simulink model "Controller_test"  (R2025b)
settings: Solver=FixedStepDiscrete  StartTime=0.0  StopTime=3*tHold  FixedStep=Ts  RelTol=1e-3
PreLoadFcn:
  | controller_params
InitFcn:
  | controller_params
undefined symbols (not defined in the file): Ao, Bo, DiscIntNeverNeededParam, K, Ke, plantD, preD, preMap, rLow, tExc, tHold, Ts, uLim, vBias, x0map, xPlant0
libraries: simulink x1
settings Model: Creator=havard  LastModifiedBy=havard

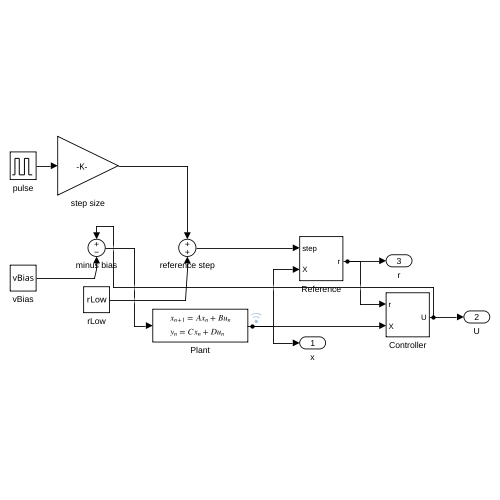
[thumbnail: Simulink's stored preview of the top-level diagram]
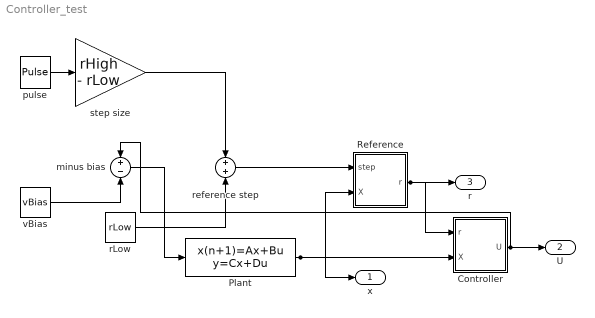
== system Controller_test ==
  Controller : Subsystem
  Plant : DiscreteStateSpace  A=plantD.A  B=plantD.B  C=plantD.C  D=0  InitialCondition=[0; xPlant0; 0; xPlant0; 0]  SampleTime=Ts
  Reference : Subsystem
  minus bias : Sum  Inputs=+-
  pulse : DiscretePulseGenerator  PulseType=Time based  Period=2*tHold  PulseWidth=50  PhaseDelay=tHold
  rLow : Constant  Value=rLow
  reference step : Sum
  step size : Gain  Gain=rHigh - rLow
  vBias : Constant  Value=vBias
  x : Outport
  U : Outport  Port=2
  r : Outport  Port=3
  wires:
  Reference/1(r) -> r/1, Controller/1(r)
  Plant/1 -> x/1, Reference/2(X), Controller/2(X)
  reference step/1 -> Reference/1(step)
  minus bias/1 -> Plant/1
  rLow/1 -> reference step/2
  step size/1 -> reference step/1
  vBias/1 -> minus bias/2
  pulse/1 -> step size/1
  Controller/1(U) -> minus bias/1, U/1

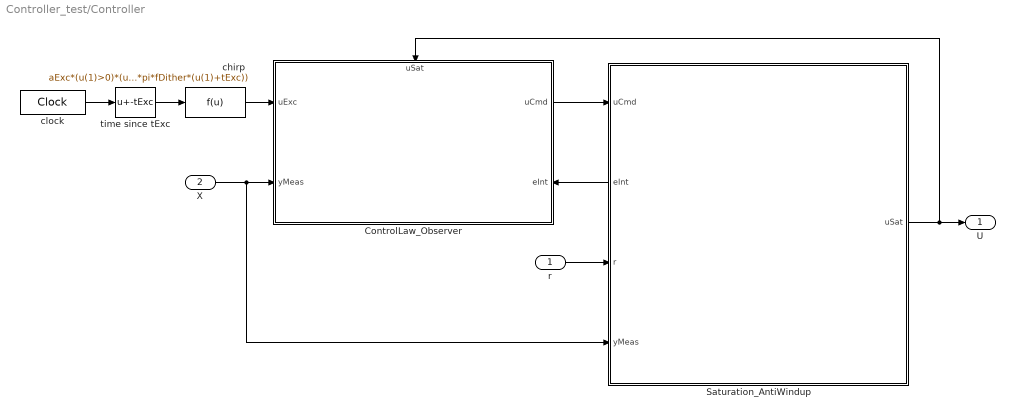
== system Controller_test/Controller ==
  r : Inport
  X : Inport  Port=2
  ControlLaw_Observer : Subsystem
      settings: PortSchema="{\"entries\":[{\"content\":{\"sides\":[{\"content\":{\"connectorIds\":[\"In1\",\"In2\"]},\"type\":\"ConnectorPlacement.EquallySpacedRectSide\",\"uuid\":\"4ab0fcb8-52c7-4a4e-9377-be86be06758b\"},{\"content\":{\"connectorIds\":[\"Out1\",\"In4\"],\"side\":\"RIGHT\"},\"type\":\"ConnectorPlacement.EquallySpacedRectSide\",\"uuid\":\"0c93ed77-db89-4914-8ed3-cc59a8eb3b85\"},{\"content\":{\"connectorIds\":[\"In3\"],\"side\":\"TOP\"},\"type\":\"ConnectorPlacement.EquallySpacedRectSide\",\"uuid\":\"1c748175-366b-4d57-8d03-3856bbcdfb09\"},{\"content\":{\"side\":\"BOTTOM\"},\"type\":\"ConnectorPlacement.EquallySpacedRectSide\",\"uuid\":\"18ee6780-29bb-4133-baad-5bb614cd70f7\"}]},\"type\":\"ConnectorPlacement.EquallySpacedConnector\",\"uuid\":\"9b829baf-7a37-4ed0-ad0c-dec2a53cf1cf\"}],\"packageUris\":[\"http://schema.mathworks.com/mf0/Connector/R2020b\"],\"version\":\"1.0\"}"
  Saturation_AntiWindup : Subsystem
      settings: PortSchema="{\"entries\":[{\"content\":{\"sides\":[{\"content\":{\"connectorIds\":[\"In1\",\"Out2\",\"In2\",\"In3\"]},\"type\":\"ConnectorPlacement.EquallySpacedRectSide\",\"uuid\":\"fd51be67-1b16-4c80-8941-43d479349b34\"},{\"content\":{\"connectorIds\":[\"Out1\"],\"side\":\"RIGHT\"},\"type\":\"ConnectorPlacement.EquallySpacedRectSide\",\"uuid\":\"50a9a10a-2e08-446e-b14e-5678e3c6d1e3\"},{\"content\":{\"side\":\"TOP\"},\"type\":\"ConnectorPlacement.EquallySpacedRectSide\",\"uuid\":\"8fd36ea3-ab38-479f-a719-6e347c4892f4\"}]},\"type\":\"ConnectorPlacement.EquallySpacedConnector\",\"uuid\":\"95e37cf3-826c-49dc-833f-2565447af58e\"}],\"packageUris\":[\"http://schema.mathworks.com/mf0/Connector/R2020b\"],\"version\":\"1.0\"}"
  chirp : Fcn  Expr=aExc*(u(1)>0)*(u(1)<tExcDur)*sin(2*pi*(fExc1*u(1) + (fExc2-fExc1)/(2*tExcDur)*u(1)^2)) + aDither*sin(2*pi*fDither*(u(1)+tExc))
  clock : DigitalClock  SampleTime=Ts
  time since tExc : Bias  Bias=-tExc  SaturateOnIntegerOverflow=off
  U : Outport
  wires:
  time since tExc/1 -> chirp/1
  clock/1 -> time since tExc/1
  chirp/1 -> ControlLaw_Observer/1(uExc)
  Saturation_AntiWindup/2(eInt) -> ControlLaw_Observer/4(eInt)
  Saturation_AntiWindup/1(uSat) -> ControlLaw_Observer/3(uSat), U/1
  ControlLaw_Observer/1(uCmd) -> Saturation_AntiWindup/1(uCmd)
  X/1 -> Saturation_AntiWindup/3(yMeas), ControlLaw_Observer/2(yMeas)
  r/1 -> Saturation_AntiWindup/2(r)

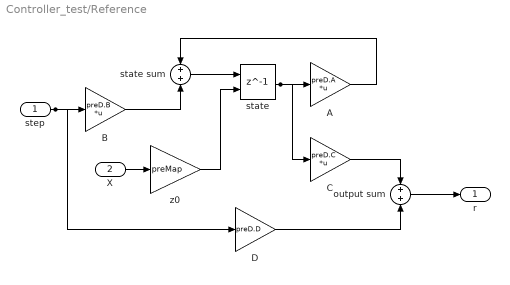
== system Controller_test/Reference ==
  step : Inport
  X : Inport  Port=2
  A : Gain  Gain=preD.A  Multiplication=Matrix(K*u)
  B : Gain  Gain=preD.B  Multiplication=Matrix(K*u)
  C : Gain  Gain=preD.C  Multiplication=Matrix(K*u)
  D : Gain  Gain=preD.D
  output sum : Sum
  state : Delay  DelayLength=1  InitialConditionSource=Input port  SampleTime=Ts
      settings: InputPortMap=u0,p4
  state sum : Sum
  z0 : Gain  Gain=preMap
  r : Outport
  wires:
  output sum/1 -> r/1
  C/1 -> output sum/1
  A/1 -> state sum/1
  D/1 -> output sum/2
  state sum/1 -> state/1
  z0/1 -> state/2
  X/1 -> z0/1
  B/1 -> state sum/2
  state/1 -> C/1, A/1
  step/1 -> B/1, D/1

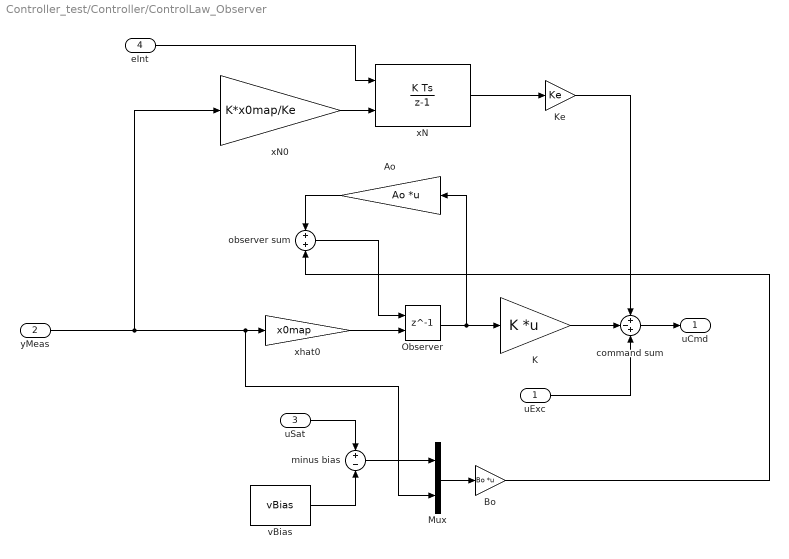
== system Controller_test/Controller/ControlLaw_Observer ==
  uExc : Inport
  yMeas : Inport  Port=2
  uSat : Inport  Port=3
  eInt : Inport  Port=4
  Ao : Gain  Gain=Ao  Multiplication=Matrix(K*u)
  Bo : Gain  Gain=Bo  Multiplication=Matrix(K*u)
  K : Gain  Gain=K  Multiplication=Matrix(K*u)
  Ke : Gain  Gain=Ke
  Mux : Mux  Inputs=2
  Observer : Delay  DelayLength=1  InitialConditionSource=Input port  SampleTime=Ts
      settings: InputPortMap=u0,p4
  command sum : Sum  Inputs=+-+
  minus bias : Sum  Inputs=+-
  observer sum : Sum
  vBias : Constant  Value=vBias
  xN : DiscreteIntegrator  InitialConditionSource=external  SampleTime=Ts  ICPrevOutput=DiscIntNeverNeededParam  ICPrevScaledInput=DiscIntNeverNeededParam
  xN0 : Gain  Gain=K*x0map/Ke
  xhat0 : Gain  Gain=x0map
  uCmd : Outport
  wires:
  Bo/1 -> observer sum/2
  Mux/1 -> Bo/1
  minus bias/1 -> Mux/1
  vBias/1 -> minus bias/2
  uSat/1 -> minus bias/1
  observer sum/1 -> Observer/1
  K/1 -> command sum/2
  xN/1 -> Ke/1
  Ao/1 -> observer sum/1
  xN0/1 -> xN/2
  uExc/1 -> command sum/3
  Observer/1 -> K/1, Ao/1
  command sum/1 -> uCmd/1
  yMeas/1 -> xN0/1, Mux/2, xhat0/1
  xhat0/1 -> Observer/2
  eInt/1 -> xN/1
  Ke/1 -> command sum/1

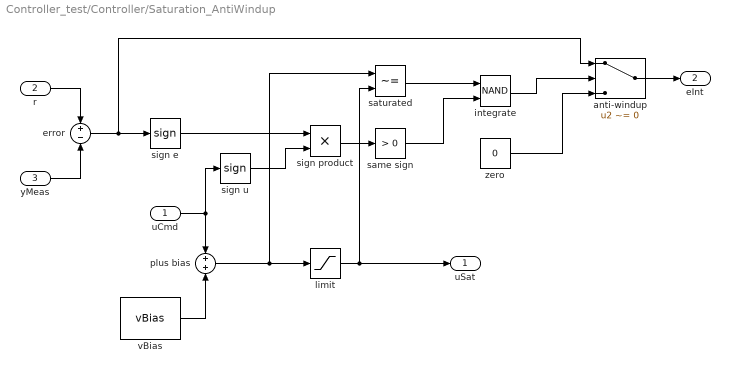
== system Controller_test/Controller/Saturation_AntiWindup ==
  uCmd : Inport
  r : Inport  Port=2
  yMeas : Inport  Port=3
  anti-windup : Switch  Criteria=u2 ~= 0  SaturateOnIntegerOverflow=off  InputSameDT=off
  error : Sum  Inputs=+-
  integrate : Logic  Operator=NAND  AllPortsSameDT=off  OutDataTypeStr=boolean
  limit : Saturate  UpperLimit=uLim(2)  LowerLimit=uLim(1)
  plus bias : Sum
  same sign : simulink/Logic and Bit Operations/Compare To Constant  relop=>  const=0  OutDataTypeStr=boolean
  saturated : RelationalOperator  Operator=~=  OutDataTypeStr=boolean  RndMeth=Simplest  InputSameDT=off
  sign e : Signum
  sign product : Product
  sign u : Signum
  vBias : Constant  Value=vBias
  zero : Constant  Value=0
  uSat : Outport
  eInt : Outport  Port=2
  wires:
  vBias/1 -> plus bias/2
  limit/1 -> uSat/1, saturated/2
  zero/1 -> anti-windup/3
  error/1 -> anti-windup/1, sign e/1
  sign e/1 -> sign product/1
  plus bias/1 -> saturated/1, limit/1
  r/1 -> error/1
  sign product/1 -> same sign/1
  uCmd/1 -> sign u/1, plus bias/1
  anti-windup/1 -> eInt/1
  saturated/1 -> integrate/1
  yMeas/1 -> error/2
  integrate/1 -> anti-windup/2
  sign u/1 -> sign product/2
  same sign/1 -> integrate/2
